simulink model "gm_PMLSM_FOC_FixedPoint_vnl"  (R2026b)
settings: Solver=FixedStepDiscrete  StopTime=0.0063  FixedStep=2e-08
undefined symbols (not defined in the file): FOC_Fixed_Config, Lookup, Ts_ACR
libraries: hdlmdlgenlib x38, simulink x16, mcbeeMathTransformLib x2
(part 1 of 6)
settings Model: Creator=lww  LastModifiedBy=lww
settings DataIOCC: ExternalInput=M3_HDL_Stimulus  LoadExternalInput=on
settings OptimizationCC: BlockReduction=off  ConditionallyExecuteInputs=off  DefaultParameterBehavior=Inlined
settings DebuggingCC: FixptConstOverflowMsg=error  InheritedTsInSrcMsg=none  IntegerOverflowMsg=error  IntegerSaturationMsg=error

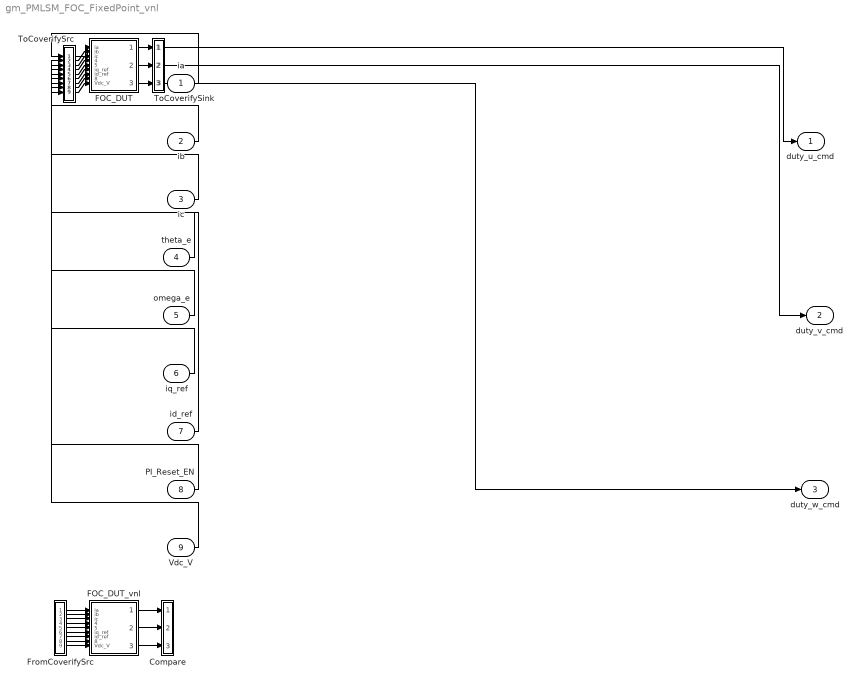
== system gm_PMLSM_FOC_FixedPoint_vnl ==
  ia : Inport  OutDataTypeStr=FOC_Fixed_Config.Types.Current  SampleTime=Ts_ACR  Interpolate=off
  ib : Inport  Port=2  OutDataTypeStr=FOC_Fixed_Config.Types.Current  SampleTime=Ts_ACR  Interpolate=off
  ic : Inport  Port=3  OutDataTypeStr=FOC_Fixed_Config.Types.Current  SampleTime=Ts_ACR  Interpolate=off
  theta_e : Inport  Port=4  OutDataTypeStr=FOC_Fixed_Config.Types.Angle  SampleTime=Ts_ACR  Interpolate=off
  omega_e : Inport  Port=5  OutDataTypeStr=FOC_Fixed_Config.Types.Omega  SampleTime=Ts_ACR  Interpolate=off
  iq_ref : Inport  Port=6  OutDataTypeStr=FOC_Fixed_Config.Types.Current  SampleTime=Ts_ACR  Interpolate=off
  id_ref : Inport  Port=7  OutDataTypeStr=FOC_Fixed_Config.Types.Current  SampleTime=Ts_ACR  Interpolate=off
  PI_Reset_EN : Inport  Port=8  OutDataTypeStr=boolean  SampleTime=Ts_ACR  Interpolate=off
  Vdc_V : Inport  Port=9  OutDataTypeStr=FOC_Fixed_Config.Types.Bus  SampleTime=Ts_ACR  Interpolate=off
  Compare : Subsystem
      mask Display: disp('')
  FOC_DUT : Subsystem
  FOC_DUT_vnl : Subsystem  TreatAsAtomicUnit=on
  FromCoverifySrc : Subsystem
      mask Display: disp('')
  ToCoverifySink : Subsystem
      mask Display: disp('')
  ToCoverifySrc : Subsystem
      mask Display: disp('')
  duty_u_cmd : Outport  OutDataTypeStr=FOC_Fixed_Config.Types.Duty
  duty_v_cmd : Outport  Port=2  OutDataTypeStr=FOC_Fixed_Config.Types.Duty
  duty_w_cmd : Outport  Port=3  OutDataTypeStr=FOC_Fixed_Config.Types.Duty
  wires:
  ToCoverifySrc/1(out1) -> FOC_DUT/1(ia)
  ToCoverifySrc/2(out2) -> FOC_DUT/2(ib)
  ToCoverifySrc/3(out3) -> FOC_DUT/3(ic)
  ToCoverifySrc/4(out4) -> FOC_DUT/4(theta_e)
  ToCoverifySrc/5(out5) -> FOC_DUT/5(omega_e)
  ToCoverifySrc/6(out6) -> FOC_DUT/6(iq_ref)
  ToCoverifySrc/7(out7) -> FOC_DUT/7(id_ref)
  ToCoverifySrc/8(out8) -> FOC_DUT/8(PI_Reset_EN)
  ToCoverifySrc/9(out9) -> FOC_DUT/9(Vdc_V)
  FOC_DUT/1(duty_u_cmd) -> ToCoverifySink/1(in1)
  FOC_DUT/2(duty_v_cmd) -> ToCoverifySink/2(in2)
  FOC_DUT/3(duty_w_cmd) -> ToCoverifySink/3(in3)
  ia/1 -> ToCoverifySrc/1(in1)
  ib/1 -> ToCoverifySrc/2(in2)
  ic/1 -> ToCoverifySrc/3(in3)
  theta_e/1 -> ToCoverifySrc/4(in4)
  omega_e/1 -> ToCoverifySrc/5(in5)
  iq_ref/1 -> ToCoverifySrc/6(in6)
  id_ref/1 -> ToCoverifySrc/7(in7)
  PI_Reset_EN/1 -> ToCoverifySrc/8(in8)
  Vdc_V/1 -> ToCoverifySrc/9(in9)
  ToCoverifySink/1(out1) -> duty_u_cmd/1
  ToCoverifySink/2(out2) -> duty_v_cmd/1
  ToCoverifySink/3(out3) -> duty_w_cmd/1
  FromCoverifySrc/1(out1) -> FOC_DUT_vnl/1(ia)
  FromCoverifySrc/2(out2) -> FOC_DUT_vnl/2(ib)
  FromCoverifySrc/3(out3) -> FOC_DUT_vnl/3(ic)
  FromCoverifySrc/4(out4) -> FOC_DUT_vnl/4(theta_e)
  FromCoverifySrc/5(out5) -> FOC_DUT_vnl/5(omega_e)
  FromCoverifySrc/6(out6) -> FOC_DUT_vnl/6(iq_ref)
  FromCoverifySrc/7(out7) -> FOC_DUT_vnl/7(id_ref)
  FromCoverifySrc/8(out8) -> FOC_DUT_vnl/8(PI_Reset_EN)
  FromCoverifySrc/9(out9) -> FOC_DUT_vnl/9(Vdc_V)
  FOC_DUT_vnl/1(duty_u_cmd) -> Compare/1(in1)
  FOC_DUT_vnl/2(duty_v_cmd) -> Compare/2(in2)
  FOC_DUT_vnl/3(duty_w_cmd) -> Compare/3(in3)

== system gm_PMLSM_FOC_FixedPoint_vnl/Compare ==
  in1 : Inport
  in2 : Inport  Port=2
  in3 : Inport  Port=3
  Assert_duty_u_cmd : Subsystem
  Assert_duty_v_cmd : Subsystem
  Assert_duty_w_cmd : Subsystem
  CleanupScopes : Subsystem
      settings: OpenFcn=|
      | blkName = gcb; %self block
      | idx = regexp(blkName, '/CleanupScopes$', 'once');
      | blkParent = blkName(1:idx-1);
      | blks=find_system(blkParent, 'LookUnderMasks', 'all','blocktype', 'Scope');
      | for itr = 1:length(blks)
      | 	 hScopeCfg = get_param(blks{itr},'ScopeConfiguration');
      | 	 hScopeCfg.Visible = ~ hScopeCfg.Visible;
      | end
      | drawnow;
      mask Display: fprintf(message('hdlcoder:cosim:vnl_dblclick').getString());
  Enable : Subsystem
      settings: OpenFcn=|
      | blkName = gcb;
      | idx = regexp(blkName, '/Enable$', 'once');
      | blkParent = blkName(1:idx-1);
      | blks=find_system(blkParent, 'LookUnderMasks', 'all','blocktype', 'Assertion');
      | e = get_param(blks{1}, 'Enabled');
      | if strcmp(e, 'on'), f= 'off';, else, f = 'on';, end
      | for ii=1:length(blks), set_param(blks{ii}, 'Enabled', f);, end
      | set_param(gcb, 'MaskDisplay',['fprintf(message(''hdlcoder:cosim:vnl_dblclick_assertions'',','''',upper(e),'''',').getString())']);
      mask Display: fprintf(message('hdlcoder:cosim:vnl_dblclick_assertions','OFF').getString());
  pathdelay1 : Delay  DelayLength=1
  pathdelay2 : Delay  DelayLength=1
  pathdelay3 : Delay  DelayLength=1
  wires:
  in1/1 -> pathdelay1/1
  pathdelay1/1 -> Assert_duty_u_cmd/1(cosim)
  [out1] -> Assert_duty_u_cmd/2(dut)
  in2/1 -> pathdelay2/1
  pathdelay2/1 -> Assert_duty_v_cmd/1(cosim)
  [out2] -> Assert_duty_v_cmd/2(dut)
  in3/1 -> pathdelay3/1
  pathdelay3/1 -> Assert_duty_w_cmd/1(cosim)
  [out3] -> Assert_duty_w_cmd/2(dut)

== system gm_PMLSM_FOC_FixedPoint_vnl/FOC_DUT ==
  ia : Inport  OutDataTypeStr=fixdt(1, 32, 24)  PortDimensions=1  SampleTime=0.0001
  ib : Inport  Port=2  OutDataTypeStr=fixdt(1, 32, 24)  PortDimensions=1  SampleTime=0.0001
  ic : Inport  Port=3  OutDataTypeStr=fixdt(1, 32, 24)  PortDimensions=1  SampleTime=0.0001
  theta_e : Inport  Port=4  OutDataTypeStr=fixdt(1, 40, 32)  PortDimensions=1  SampleTime=0.0001
  omega_e : Inport  Port=5  OutDataTypeStr=fixdt(1, 40, 24)  PortDimensions=1  SampleTime=0.0001
  iq_ref : Inport  Port=6  OutDataTypeStr=fixdt(1, 32, 24)  PortDimensions=1  SampleTime=0.0001
  id_ref : Inport  Port=7  OutDataTypeStr=fixdt(1, 32, 24)  PortDimensions=1  SampleTime=0.0001
  PI_Reset_EN : Inport  Port=8  OutDataTypeStr=boolean  PortDimensions=1  SampleTime=0.0001
  Vdc_V : Inport  Port=9  OutDataTypeStr=fixdt(0, 32, 24)  PortDimensions=1  SampleTime=0.0001
  FOC_DUT : Subsystem  TreatAsAtomicUnit=on
  t : RateTransition  OutPortSampleTimeOpt=Multiple of input port sample time  OutPortSampleTimeMultiple=5000
  t1 : RateTransition  OutPortSampleTimeOpt=Multiple of input port sample time  OutPortSampleTimeMultiple=5000
  t2 : RateTransition  OutPortSampleTimeOpt=Multiple of input port sample time  OutPortSampleTimeMultiple=5000
  duty_u_cmd : Outport  OutDataTypeStr=fixdt(0, 32, 30)  PortDimensions=1  SampleTime=0.0001
  duty_v_cmd : Outport  Port=2  OutDataTypeStr=fixdt(0, 32, 30)  PortDimensions=1  SampleTime=0.0001
  duty_w_cmd : Outport  Port=3  OutDataTypeStr=fixdt(0, 32, 30)  PortDimensions=1  SampleTime=0.0001
  wires:
  t2/1 -> duty_w_cmd/1
  t1/1 -> duty_v_cmd/1
  t/1 -> duty_u_cmd/1
  FOC_DUT/3(duty_w_cmd) -> t2/1
  FOC_DUT/1(duty_u_cmd) -> t/1
  Vdc_V/1 -> FOC_DUT/9(Vdc_V)
  FOC_DUT/2(duty_v_cmd) -> t1/1
  PI_Reset_EN/1 -> FOC_DUT/8(PI_Reset_EN)
  ib/1 -> FOC_DUT/2(ib)
  ia/1 -> FOC_DUT/1(ia)
  ic/1 -> FOC_DUT/3(ic)
  theta_e/1 -> FOC_DUT/4(theta_e)
  omega_e/1 -> FOC_DUT/5(omega_e)
  iq_ref/1 -> FOC_DUT/6(iq_ref)
  id_ref/1 -> FOC_DUT/7(id_ref)

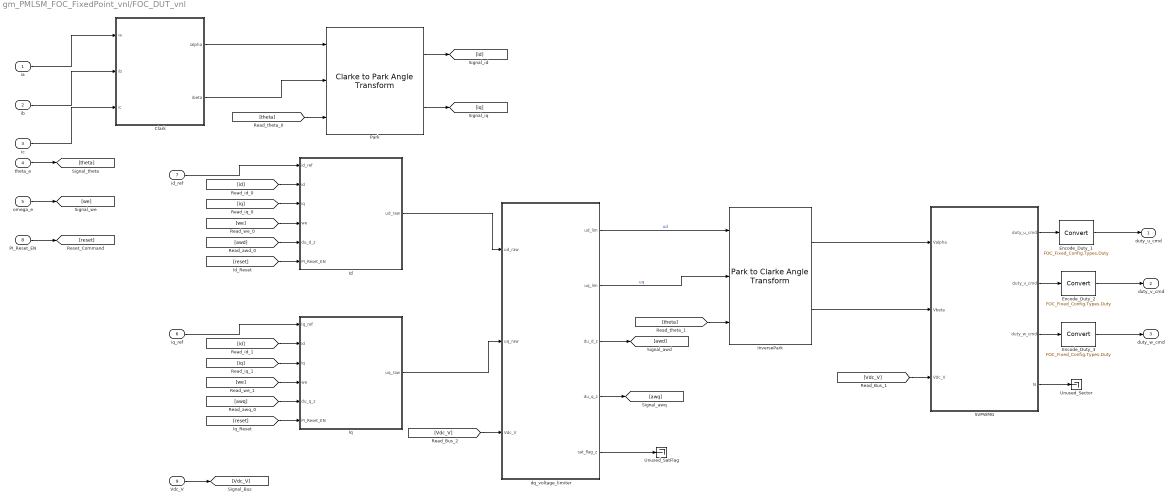
== system gm_PMLSM_FOC_FixedPoint_vnl/FOC_DUT_vnl ==
  ia : Inport
  ib : Inport  Port=2
  ic : Inport  Port=3
  theta_e : Inport  Port=4
  omega_e : Inport  Port=5
  iq_ref : Inport  Port=6
  id_ref : Inport  Port=7
  PI_Reset_EN : Inport  Port=8
  Vdc_V : Inport  Port=9
  Clark : Subsystem  TreatAsAtomicUnit=on  RTWFcnName=Clack_Fun
      settings: RTWFcnNameOpts=User specified
  Encode_Duty_1 : DataTypeConversion  OutDataTypeStr=FOC_Fixed_Config.Types.Duty  RndMeth=Convergent
  Encode_Duty_2 : DataTypeConversion  OutDataTypeStr=FOC_Fixed_Config.Types.Duty  RndMeth=Convergent
  Encode_Duty_3 : DataTypeConversion  OutDataTypeStr=FOC_Fixed_Config.Types.Duty  RndMeth=Convergent
  Id : Subsystem  TreatAsAtomicUnit=on  RTWFcnName=Id_Fun
      settings: RTWFcnNameOpts=User specified
  InversePark : mcbeeMathTransformLib/Park to Clarke Angle Transform  AxisAlignment=D-axis  UseWithEmbedded=on  PhaseInput=Two inputs  ThetaInput=Electrical position  AngleInput=Radians  N_points=1024
      settings: LibrarySourceBlock=mcbhdllib/Controls/Math Transforms/Inverse Park Transform
  Iq : Subsystem  TreatAsAtomicUnit=on  RTWFcnName=Iq_Fun
      settings: RTWFcnNameOpts=User specified
  Park : mcbeeMathTransformLib/Clarke to Park Angle Transform  AxisAlignment=D-axis  UseWithEmbedded=on  PhaseInput=Two inputs  ThetaInput=Electrical position  AngleInput=Radians  N_points=1024
      settings: LibrarySourceBlock=mcblib/Controls/Math Transforms/Park Transform
  SVPWMG : Subsystem  TreatAsAtomicUnit=on  RTWFcnName=SVPWM_Gen_Fun
      settings: RTWFcnNameOpts=User specified
  Unused_SatFlag : Terminator
  Unused_Sector : Terminator
  dq_voltage_limiter : Subsystem
  duty_u_cmd : Outport
  duty_v_cmd : Outport  Port=2
  duty_w_cmd : Outport  Port=3
  wires:
  dq_voltage_limiter/3(du_d_z) -> [awd]
  dq_voltage_limiter/5(sat_flag_z) -> Unused_SatFlag/1
  dq_voltage_limiter/4(du_q_z) -> [awq]
  dq_voltage_limiter/2(uq_lim) -> InversePark/2  "uq"
  dq_voltage_limiter/1(ud_lim) -> InversePark/1  "ud"
  SVPWMG/4("N ") -> Unused_Sector/1
  SVPWMG/3(duty_w_cmd) -> Encode_Duty_3/1
  SVPWMG/2(duty_v_cmd) -> Encode_Duty_2/1
  SVPWMG/1(duty_u_cmd) -> Encode_Duty_1/1
  [we] -> Iq/4(we)
  [we] -> Id/4(we)
  [theta] -> InversePark/3
  [theta] -> Park/3
  [iq] -> Iq/3(iq)
  [iq] -> Id/3(iq)
  [id] -> Iq/2(id)
  [id] -> Id/2(id)
  [awq] -> Iq/5(du_q_z)
  [awd] -> Id/5(du_d_z)
  [Vdc_V] -> dq_voltage_limiter/3(Vdc_V)
  [Vdc_V] -> SVPWMG/3(Vdc_V)
  Park/2 -> [iq]
  Park/1 -> [id]
  [reset] -> Iq/6(PI_Reset_EN)
  Iq/1(uq_raw) -> dq_voltage_limiter/2(uq_raw)
  InversePark/2 -> SVPWMG/2(Vbeta)
  InversePark/1 -> SVPWMG/1(Valpha)
  [reset] -> Id/6(PI_Reset_EN)
  Id/1(ud_raw) -> dq_voltage_limiter/1(ud_raw)
  Encode_Duty_3/1 -> duty_w_cmd/1
  Encode_Duty_2/1 -> duty_v_cmd/1
  Encode_Duty_1/1 -> duty_u_cmd/1
  Clark/2(ibeta) -> Park/2
  Clark/1(ialpha) -> Park/1
  Vdc_V/1 -> [Vdc_V]
  PI_Reset_EN/1 -> [reset]
  id_ref/1 -> Id/1(id_ref)
  iq_ref/1 -> Iq/1(Iq_ref)
  omega_e/1 -> [we]
  theta_e/1 -> [theta]
  ic/1 -> Clark/3(ic)
  ib/1 -> Clark/2(ib)
  ia/1 -> Clark/1(ia)

== system gm_PMLSM_FOC_FixedPoint_vnl/FromCoverifySrc ==
  out1 : Outport
  out2 : Outport  Port=2
  out3 : Outport  Port=3
  out4 : Outport  Port=4
  out5 : Outport  Port=5
  out6 : Outport  Port=6
  out7 : Outport  Port=7
  out8 : Outport  Port=8
  out9 : Outport  Port=9
  wires:
  [in1] -> out1/1
  [in2] -> out2/1
  [in3] -> out3/1
  [in4] -> out4/1
  [in5] -> out5/1
  [in6] -> out6/1
  [in7] -> out7/1
  [in8] -> out8/1
  [in9] -> out9/1

== system gm_PMLSM_FOC_FixedPoint_vnl/ToCoverifySink ==
  in1 : Inport
  in2 : Inport  Port=2
  in3 : Inport  Port=3
  out1 : Outport
  out2 : Outport  Port=2
  out3 : Outport  Port=3
  tag scope: out1=global, out2=global, out3=global
  wires:
  in1/1 -> out1/1, [out1]
  in2/1 -> out2/1, [out2]
  in3/1 -> out3/1, [out3]

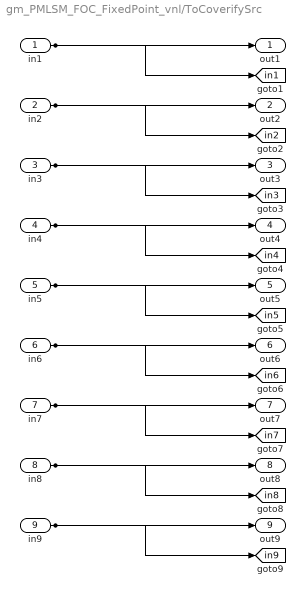
== system gm_PMLSM_FOC_FixedPoint_vnl/ToCoverifySrc ==
  in1 : Inport
  in2 : Inport  Port=2
  in3 : Inport  Port=3
  in4 : Inport  Port=4
  in5 : Inport  Port=5
  in6 : Inport  Port=6
  in7 : Inport  Port=7
  in8 : Inport  Port=8
  in9 : Inport  Port=9
  out1 : Outport
  out2 : Outport  Port=2
  out3 : Outport  Port=3
  out4 : Outport  Port=4
  out5 : Outport  Port=5
  out6 : Outport  Port=6
  out7 : Outport  Port=7
  out8 : Outport  Port=8
  out9 : Outport  Port=9
  tag scope: in1=global, in2=global, in3=global, in4=global, in5=global, in6=global, in7=global, in8=global, in9=global
  wires:
  in1/1 -> out1/1, [in1]
  in2/1 -> out2/1, [in2]
  in3/1 -> out3/1, [in3]
  in4/1 -> out4/1, [in4]
  in5/1 -> out5/1, [in5]
  in6/1 -> out6/1, [in6]
  in7/1 -> out7/1, [in7]
  in8/1 -> out8/1, [in8]
  in9/1 -> out9/1, [in9]

== system gm_PMLSM_FOC_FixedPoint_vnl/Compare/Assert_duty_u_cmd ==
  cosim : Inport
  dut : Inport  Port=2
  AssertEq : Assertion  StopWhenAssertionFail=off
  Compare To Zero : simulink/Logic and Bit Operations/Compare To Zero  relop===  OutDataTypeStr=boolean
  Constant1 : Constant  Value=0  OutDataTypeStr=fixdt(0, 32, 30)  SampleTime=-1
  Counter : simulink/Sources/Counter Free-Running  NumBits=32  tsamp=-1
  IgnoreCycles : Constant  Value=2  SampleTime=-1
  Relational Operator : RelationalOperator  Operator=<  OutDataTypeStr=boolean  InputSameDT=off
  Relational Operator1 : RelationalOperator  Operator===  OutDataTypeStr=boolean  InputSameDT=off
  Switch : Switch  Criteria=u2 ~= 0  SaturateOnIntegerOverflow=off  InputSameDT=off
  Switch1 : Switch  Criteria=u2 ~= 0  SaturateOnIntegerOverflow=off  InputSameDT=off
  compare: duty_u_cmd : Scope  NumInputPorts=3
      settings: ActiveDisplayYMinimum=-5  ActiveDisplayYMaximum=5  DataLoggingVariableName=ScopeData3
  wires:
  Compare To Zero/1 -> compare: duty_u_cmd/3  "err"
  Relational Operator1/1 -> Compare To Zero/1, AssertEq/1
  Switch1/1 -> compare: duty_u_cmd/1, Relational Operator1/1
  Switch/1 -> compare: duty_u_cmd/2, Relational Operator1/2
  Constant1/1 -> Switch/1, Switch1/1
  Relational Operator/1 -> Switch/2, Switch1/2
  cosim/1 -> Switch1/3  "cosim"
  dut/1 -> Switch/3  "dut ref"
  Counter/1 -> Relational Operator/1
  IgnoreCycles/1 -> Relational Operator/2

== system gm_PMLSM_FOC_FixedPoint_vnl/Compare/Assert_duty_v_cmd ==
  cosim : Inport
  dut : Inport  Port=2
  AssertEq : Assertion  StopWhenAssertionFail=off
  Compare To Zero : simulink/Logic and Bit Operations/Compare To Zero  relop===  OutDataTypeStr=boolean
  Constant1 : Constant  Value=0  OutDataTypeStr=fixdt(0, 32, 30)  SampleTime=-1
  Counter : simulink/Sources/Counter Free-Running  NumBits=32  tsamp=-1
  IgnoreCycles : Constant  Value=2  SampleTime=-1
  Relational Operator : RelationalOperator  Operator=<  OutDataTypeStr=boolean  InputSameDT=off
  Relational Operator1 : RelationalOperator  Operator===  OutDataTypeStr=boolean  InputSameDT=off
  Switch : Switch  Criteria=u2 ~= 0  SaturateOnIntegerOverflow=off  InputSameDT=off
  Switch1 : Switch  Criteria=u2 ~= 0  SaturateOnIntegerOverflow=off  InputSameDT=off
  compare: duty_v_cmd : Scope  NumInputPorts=3
      settings: ActiveDisplayYMinimum=-5  ActiveDisplayYMaximum=5  DataLoggingVariableName=ScopeData3
  wires:
  Compare To Zero/1 -> compare: duty_v_cmd/3  "err"
  Relational Operator1/1 -> Compare To Zero/1, AssertEq/1
  Switch1/1 -> compare: duty_v_cmd/1, Relational Operator1/1
  Switch/1 -> compare: duty_v_cmd/2, Relational Operator1/2
  Constant1/1 -> Switch/1, Switch1/1
  Relational Operator/1 -> Switch/2, Switch1/2
  cosim/1 -> Switch1/3  "cosim"
  dut/1 -> Switch/3  "dut ref"
  Counter/1 -> Relational Operator/1
  IgnoreCycles/1 -> Relational Operator/2

== system gm_PMLSM_FOC_FixedPoint_vnl/Compare/Assert_duty_w_cmd ==
  cosim : Inport
  dut : Inport  Port=2
  AssertEq : Assertion  StopWhenAssertionFail=off
  Compare To Zero : simulink/Logic and Bit Operations/Compare To Zero  relop===  OutDataTypeStr=boolean
  Constant1 : Constant  Value=0  OutDataTypeStr=fixdt(0, 32, 30)  SampleTime=-1
  Counter : simulink/Sources/Counter Free-Running  NumBits=32  tsamp=-1
  IgnoreCycles : Constant  Value=2  SampleTime=-1
  Relational Operator : RelationalOperator  Operator=<  OutDataTypeStr=boolean  InputSameDT=off
  Relational Operator1 : RelationalOperator  Operator===  OutDataTypeStr=boolean  InputSameDT=off
  Switch : Switch  Criteria=u2 ~= 0  SaturateOnIntegerOverflow=off  InputSameDT=off
  Switch1 : Switch  Criteria=u2 ~= 0  SaturateOnIntegerOverflow=off  InputSameDT=off
  compare: duty_w_cmd : Scope  NumInputPorts=3
      settings: ActiveDisplayYMinimum=-5  ActiveDisplayYMaximum=5  DataLoggingVariableName=ScopeData3
  wires:
  Compare To Zero/1 -> compare: duty_w_cmd/3  "err"
  Relational Operator1/1 -> Compare To Zero/1, AssertEq/1
  Switch1/1 -> compare: duty_w_cmd/1, Relational Operator1/1
  Switch/1 -> compare: duty_w_cmd/2, Relational Operator1/2
  Constant1/1 -> Switch/1, Switch1/1
  Relational Operator/1 -> Switch/2, Switch1/2
  cosim/1 -> Switch1/3  "cosim"
  dut/1 -> Switch/3  "dut ref"
  Counter/1 -> Relational Operator/1
  IgnoreCycles/1 -> Relational Operator/2

== system gm_PMLSM_FOC_FixedPoint_vnl/Compare/CleanupScopes ==

== system gm_PMLSM_FOC_FixedPoint_vnl/Compare/Enable ==

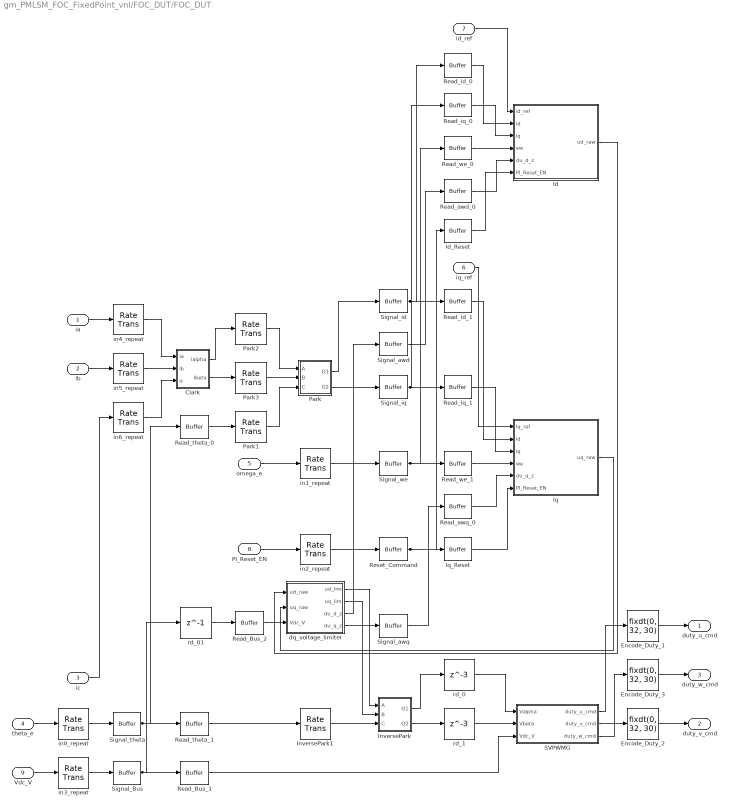
== system gm_PMLSM_FOC_FixedPoint_vnl/FOC_DUT/FOC_DUT ==
  ia : Inport  OutDataTypeStr=fixdt(1,32,24,'DataTypeOverride', 'Off')  PortDimensions=1  SampleTime=0.0001
  ib : Inport  Port=2  OutDataTypeStr=fixdt(1,32,24,'DataTypeOverride', 'Off')  PortDimensions=1  SampleTime=0.0001
  ic : Inport  Port=3  OutDataTypeStr=fixdt(1,32,24,'DataTypeOverride', 'Off')  PortDimensions=1  SampleTime=0.0001
  theta_e : Inport  Port=4  OutDataTypeStr=fixdt(1,40,32,'DataTypeOverride', 'Off')  PortDimensions=1  SampleTime=0.0001
  omega_e : Inport  Port=5  OutDataTypeStr=fixdt(1,40,24,'DataTypeOverride', 'Off')  PortDimensions=1  SampleTime=0.0001
  iq_ref : Inport  Port=6  OutDataTypeStr=fixdt(1,32,24,'DataTypeOverride', 'Off')  PortDimensions=1  SampleTime=0.0001
  id_ref : Inport  Port=7  OutDataTypeStr=fixdt(1,32,24,'DataTypeOverride', 'Off')  PortDimensions=1  SampleTime=0.0001
  PI_Reset_EN : Inport  Port=8  OutDataTypeStr=boolean  PortDimensions=1  SampleTime=0.0001
  Vdc_V : Inport  Port=9  OutDataTypeStr=fixdt(0,32,24,'DataTypeOverride', 'Off')  PortDimensions=1  SampleTime=0.0001
  Clark : Subsystem
  Encode_Duty_1 : DataTypeConversion  OutDataTypeStr=fixdt(0, 32, 30)  RndMeth=Convergent  SampleTime=2e-08
  Encode_Duty_2 : DataTypeConversion  OutDataTypeStr=fixdt(0, 32, 30)  RndMeth=Convergent  SampleTime=2e-08
  Encode_Duty_3 : DataTypeConversion  OutDataTypeStr=fixdt(0, 32, 30)  RndMeth=Convergent  SampleTime=2e-08
  Id : Subsystem
  Id_Reset : hdlmdlgenlib/Buffer
  InversePark : Subsystem  mask(Park to Clarke Angle Transform){AxisAlignment=D-axis, UseWithEmbedded=on, PhaseInput='Two inputs', ThetaInput=Electrical position, AngleInput=Radians, N_points=1024}
      mask prompts: AxisAlignment "shared_mcbeeblks:mcbeeblks:InvPBlkPrmAlign"; UseWithEmbedded "shared_mcbeeblks:mcbeeblks:BlkEmbeddedUse"; PhaseInput "shared_mcbeeblks:mcbeeblks:InvPPrmInp"; ThetaInput "shared_mcbeeblks:mcbeeblks:InvPPrmTheta"; AngleInput "shared_mcbeeblks:mcbeeblks:InvPThetaUnits"; N_points "shared_mcbeeblks:mcbeeblks:InvPPrmLUTSize"
      mask help: shared_mcbeeblks:mcbeeblks:InvPBlkDlgDes
      mask init:
      | AngleInput = 2;
      | AxisAlignment = 1;
      | N_points = 1024;
      | PhaseInput = 1;
      | ThetaInput = 1;
      | UseWithEmbedded = 1;
      mask Help: eval('mcbeeutil.mcbeesharedhelp(''inverseparktransform'')')
      mask TypeOptions AxisAlignment: shared_mcbeeblks:mcbeeblks:InvPpopDaxis | shared_mcbeeblks:mcbeeblks:InvPpopQaxis
      mask Callback UseWithEmbedded: mcbeeutil.mcbeeParkToClarkeCb('embeddeduse',gcbh);
      mask TypeOptions ThetaInput: shared_mcbeeblks:mcbeeblks:InvPPopElec | shared_mcbeeblks:mcbeeblks:InvPPopSinCos
      mask Callback ThetaInput: mcbeeutil.mcbeeParkToClarkeCb('ThetaInputCb',gcbh);
      mask TypeOptions AngleInput: shared_mcbeeblks:mcbeeblks:InvPPopPUUnit | shared_mcbeeblks:mcbeeblks:InvPPopRadUnit | shared_mcbeeblks:mcbeeblks:InvPPopDegUnit
      mask Display:
      | fprintf('Park to\nClarke')
      | port_label('input',1, 'd','interpreter', 'tex');
      | port_label('input',2, 'q','interpreter', 'tex');
      | port_label('input',3, '\theta_e','interpreter', 'tex');
      | port_label('output',1, '\alpha','interpreter', 'tex');
      | port_label('output',2, '\beta','interpreter', 'tex');
  InversePark1 : RateTransition  OutPortSampleTimeOpt=Multiple of input port sample time  OutPortSampleTimeMultiple=5000
  Iq : Subsystem
  Iq_Reset : hdlmdlgenlib/Buffer
  Park : Subsystem  mask(Clarke to Park Angle Transform){AxisAlignment=D-axis, UseWithEmbedded=on, PhaseInput='Two inputs', ThetaInput=Electrical position, AngleInput=Radians, N_points=1024}
      mask prompts: AxisAlignment "shared_mcbeeblks:mcbeeblks:ParkBlkPrmAlign"; UseWithEmbedded "shared_mcbeeblks:mcbeeblks:BlkEmbeddedUse"; PhaseInput "shared_mcbeeblks:mcbeeblks:ParkPrmInp"; ThetaInput "shared_mcbeeblks:mcbeeblks:ParkPrmTheta"; AngleInput "shared_mcbeeblks:mcbeeblks:ParkPrmThetaUnits"; N_points "shared_mcbeeblks:mcbeeblks:ParkPrmLUTSize"
      mask help: shared_mcbeeblks:mcbeeblks:ParkBlkDlgDes
      mask init:
      | AngleInput = 2;
      | AxisAlignment = 1;
      | N_points = 1024;
      | PhaseInput = 1;
      | ThetaInput = 1;
      | UseWithEmbedded = 1;
      mask Help: eval('mcbeeutil.mcbeesharedhelp(''parktransform'')')
      mask TypeOptions AxisAlignment: shared_mcbeeblks:mcbeeblks:ParkpopDaxis | shared_mcbeeblks:mcbeeblks:ParkpopQaxis
      mask Callback UseWithEmbedded: mcbeeutil.mcbeeClarkeToParkCb('embeddeduse',gcbh);
      mask TypeOptions ThetaInput: shared_mcbeeblks:mcbeeblks:ParkPopElec | shared_mcbeeblks:mcbeeblks:ParkPopSinCos
      mask Callback ThetaInput: mcbeeutil.mcbeeClarkeToParkCb('ThetaInputCb',gcbh)
      mask TypeOptions AngleInput: shared_mcbeeblks:mcbeeblks:ParkPopPUUnit | shared_mcbeeblks:mcbeeblks:ParkPopRadUnit | shared_mcbeeblks:mcbeeblks:ParkPopDegUnit
      mask Display:
      | fprintf('Clarke to\nPark')
      | port_label('input',1, '\alpha','interpreter', 'tex');
      | port_label('input',2, '\beta','interpreter', 'tex');
      | port_label('input',3, '\theta_e','interpreter', 'tex');
      | port_label('output',1, 'd','interpreter', 'tex');
      | port_label('output',2, 'q','interpreter', 'tex');
  Park1 : RateTransition  OutPortSampleTimeOpt=Multiple of input port sample time  OutPortSampleTimeMultiple=5000
  Park2 : RateTransition  OutPortSampleTimeOpt=Multiple of input port sample time  OutPortSampleTimeMultiple=5000
  Park3 : RateTransition  OutPortSampleTimeOpt=Multiple of input port sample time  OutPortSampleTimeMultiple=5000
  Read_Bus_1 : hdlmdlgenlib/Buffer
  Read_Bus_2 : hdlmdlgenlib/Buffer
  Read_awd_0 : hdlmdlgenlib/Buffer
  Read_awq_0 : hdlmdlgenlib/Buffer
  Read_id_0 : hdlmdlgenlib/Buffer
  Read_id_1 : hdlmdlgenlib/Buffer
  Read_iq_0 : hdlmdlgenlib/Buffer
  Read_iq_1 : hdlmdlgenlib/Buffer
  Read_theta_0 : hdlmdlgenlib/Buffer
  Read_theta_1 : hdlmdlgenlib/Buffer
  Read_we_0 : hdlmdlgenlib/Buffer
  Read_we_1 : hdlmdlgenlib/Buffer
  Reset_Command : hdlmdlgenlib/Buffer
  SVPWMG : Subsystem
  Signal_Bus : hdlmdlgenlib/Buffer
  Signal_awd : hdlmdlgenlib/Buffer
  Signal_awq : hdlmdlgenlib/Buffer
  Signal_id : hdlmdlgenlib/Buffer
  Signal_iq : hdlmdlgenlib/Buffer
  Signal_theta : hdlmdlgenlib/Buffer
  Signal_we : hdlmdlgenlib/Buffer
  dq_voltage_limiter : Subsystem
  in0_repeat : RateTransition  Integrity=off  Deterministic=off  OutPortSampleTimeOpt=Multiple of input port sample time  OutPortSampleTimeMultiple=1/5000
  in1_repeat : RateTransition  Integrity=off  Deterministic=off  OutPortSampleTimeOpt=Multiple of input port sample time  OutPortSampleTimeMultiple=1/5000
  in2_repeat : RateTransition  Integrity=off  Deterministic=off  OutPortSampleTimeOpt=Multiple of input port sample time  OutPortSampleTimeMultiple=1/5000
  in3_repeat : RateTransition  Integrity=off  Deterministic=off  OutPortSampleTimeOpt=Multiple of input port sample time  OutPortSampleTimeMultiple=1/5000
  in4_repeat : RateTransition  Integrity=off  Deterministic=off  OutPortSampleTimeOpt=Multiple of input port sample time  OutPortSampleTimeMultiple=1/5000
  in5_repeat : RateTransition  Integrity=off  Deterministic=off  OutPortSampleTimeOpt=Multiple of input port sample time  OutPortSampleTimeMultiple=1/5000
  in6_repeat : RateTransition  Integrity=off  Deterministic=off  OutPortSampleTimeOpt=Multiple of input port sample time  OutPortSampleTimeMultiple=1/5000
  rd_0 : Delay  DelayLength=3  InitialCondition=0  SampleTime=2e-08
  rd_01 : Delay  DelayLength=1  InitialCondition=0  SampleTime=2e-08
  rd_1 : Delay  DelayLength=3  InitialCondition=0  SampleTime=2e-08
  duty_u_cmd : Outport  OutDataTypeStr=fixdt(0,32,30,'DataTypeOverride', 'Off')  PortDimensions=1  SampleTime=2e-08
  duty_v_cmd : Outport  Port=2  OutDataTypeStr=fixdt(0,32,30,'DataTypeOverride', 'Off')  PortDimensions=1  SampleTime=2e-08
  duty_w_cmd : Outport  Port=3  OutDataTypeStr=fixdt(0,32,30,'DataTypeOverride', 'Off')  PortDimensions=1  SampleTime=2e-08
  wires:
  Encode_Duty_3/1 -> duty_w_cmd/1
  Iq/1(uq_raw) -> dq_voltage_limiter/2(uq_raw)
  Read_awq_0/1 -> Iq/5(du_q_z)
  Read_iq_1/1 -> Iq/3(iq)
  Read_id_1/1 -> Iq/2(id)
  rd_0/1 -> SVPWMG/1(Valpha)
  iq_ref/1 -> Iq/1(Iq_ref)
  Read_we_0/1 -> Id/4(we)
  Read_iq_0/1 -> Id/3(iq)
  InversePark/1(O1) -> rd_0/1
  Signal_we/1 -> Read_we_0/1, Read_we_1/1
  Signal_iq/1 -> Read_iq_0/1, Read_iq_1/1
  Signal_awd/1 -> Read_awd_0/1
  InversePark1/1 -> InversePark/3(C)
  dq_voltage_limiter/4(du_q_z) -> Signal_awq/1
  SVPWMG/1(duty_u_cmd) -> Encode_Duty_1/1
  dq_voltage_limiter/3(du_d_z) -> Signal_awd/1
  Read_we_1/1 -> Iq/4(we)
  dq_voltage_limiter/1(ud_lim) -> InversePark/1(A)
  Encode_Duty_1/1 -> duty_u_cmd/1
  in2_repeat/1 -> Reset_Command/1
  in1_repeat/1 -> Signal_we/1
  Id_Reset/1 -> Id/6(PI_Reset_EN)
  Park/2(O2) -> Signal_iq/1
  SVPWMG/2(duty_v_cmd) -> Encode_Duty_2/1
  Park/1(O1) -> Signal_id/1
  Read_Bus_2/1 -> dq_voltage_limiter/3(Vdc_V)
  id_ref/1 -> Id/1(id_ref)
  PI_Reset_EN/1 -> in2_repeat/1
  omega_e/1 -> in1_repeat/1
  Park1/1 -> Park/3(C)
  Park3/1 -> Park/2(B)
  Park2/1 -> Park/1(A)
  Iq_Reset/1 -> Iq/6(PI_Reset_EN)
  Id/1(ud_raw) -> dq_voltage_limiter/1(ud_raw)
  Read_Bus_1/1 -> SVPWMG/3(Vdc_V)
  Read_theta_1/1 -> InversePark1/1
  rd_01/1 -> Read_Bus_2/1
  Signal_awq/1 -> Read_awq_0/1
  Encode_Duty_2/1 -> duty_v_cmd/1
  Read_theta_0/1 -> Park1/1
  InversePark/2(O2) -> rd_1/1
  Clark/2(ibeta) -> Park3/1
  Read_id_0/1 -> Id/2(id)
  Clark/1(ialpha) -> Park2/1
  Signal_theta/1 -> Read_theta_1/1, Read_theta_0/1
  in6_repeat/1 -> Clark/3(ic)
  Reset_Command/1 -> Id_Reset/1, Iq_Reset/1
  rd_1/1 -> SVPWMG/2(Vbeta)
  in5_repeat/1 -> Clark/2(ib)
  in4_repeat/1 -> Clark/1(ia)
  dq_voltage_limiter/2(uq_lim) -> InversePark/2(B)
  in0_repeat/1 -> Signal_theta/1
  Read_awd_0/1 -> Id/5(du_d_z)
  ic/1 -> in6_repeat/1
  Signal_Bus/1 -> rd_01/1, Read_Bus_1/1
  SVPWMG/3(duty_w_cmd) -> Encode_Duty_3/1
  ib/1 -> in5_repeat/1
  in3_repeat/1 -> Signal_Bus/1
  Vdc_V/1 -> in3_repeat/1
  ia/1 -> in4_repeat/1
  theta_e/1 -> in0_repeat/1
  Signal_id/1 -> Read_id_0/1, Read_id_1/1

== system gm_PMLSM_FOC_FixedPoint_vnl/FOC_DUT_vnl/Clark ==
  note: alpha=(A-0.5*(B+C))*2/3
      | Beta=sqrt(3)/2*(B-C)*2/3
  ia : Inport
  ib : Inport  Port=2
  ic : Inport  Port=3
  Add : Sum  Inputs=+--  OutDataTypeStr=FOC_Fixed_Config.Types.Work  AccumDataTypeStr=FOC_Fixed_Config.Types.Work  RndMeth=Convergent  SaturateOnIntegerOverflow=on
  Add1 : Sum  Inputs=+-  OutDataTypeStr=FOC_Fixed_Config.Types.Work  AccumDataTypeStr=FOC_Fixed_Config.Types.Work  RndMeth=Convergent  SaturateOnIntegerOverflow=on
  Gain : Gain  Gain=0.5  ParamDataTypeStr=FOC_Fixed_Config.Types.Coefficient  OutDataTypeStr=FOC_Fixed_Config.Types.Work  RndMeth=Convergent  SaturateOnIntegerOverflow=on
  Gain1 : Gain  Gain=0.5  ParamDataTypeStr=FOC_Fixed_Config.Types.Coefficient  OutDataTypeStr=FOC_Fixed_Config.Types.Work  RndMeth=Convergent  SaturateOnIntegerOverflow=on
  Gain2 : Gain  Gain=FOC_Fixed_Config.Coefficients.TwoThird.quantized  ParamDataTypeStr=FOC_Fixed_Config.Types.Coefficient  OutDataTypeStr=FOC_Fixed_Config.Types.Work  RndMeth=Convergent  SaturateOnIntegerOverflow=on
  Gain3 : Gain  Gain=FOC_Fixed_Config.Coefficients.InvSqrt3.quantized  ParamDataTypeStr=FOC_Fixed_Config.Types.Coefficient  OutDataTypeStr=FOC_Fixed_Config.Types.Work  RndMeth=Convergent  SaturateOnIntegerOverflow=on
  ialpha : Outport
  ibeta : Outport  Port=2
  wires:
  Gain/1 -> Add/2
  Gain2/1 -> ialpha/1  "ialf"
  Add/1 -> Gain2/1
  Gain3/1 -> ibeta/1  "ibeta"
  ic/1 -> Gain1/1, Add1/2
  Add1/1 -> Gain3/1
  ib/1 -> Gain/1, Add1/1
  ia/1 -> Add/1
  Gain1/1 -> Add/3

== system gm_PMLSM_FOC_FixedPoint_vnl/FOC_DUT_vnl/Id ==
  note: 起到使能时初始化一下的作用
  id_ref : Inport
  id : Inport  Port=2
  iq : Inport  Port=3
  we : Inport  Port=4
  du_d_z : Inport  Port=5
  PI_Reset_EN : Inport  Port=6
  " " : Gain  Gain=FOC_Fixed_Config.Coefficients.KiTs.quantized  ParamDataTypeStr=FOC_Fixed_Config.Types.Coefficient  OutDataTypeStr=FOC_Fixed_Config.Types.Work  RndMeth=Convergent  SaturateOnIntegerOverflow=on
  "  " : Gain  Gain=FOC_Fixed_Config.Coefficients.Kp.quantized  ParamDataTypeStr=FOC_Fixed_Config.Types.Coefficient  OutDataTypeStr=FOC_Fixed_Config.Types.Work  RndMeth=Convergent  SaturateOnIntegerOverflow=on
  Add1 : Sum  OutDataTypeStr=FOC_Fixed_Config.Types.Work  AccumDataTypeStr=FOC_Fixed_Config.Types.Work  RndMeth=Convergent  SaturateOnIntegerOverflow=on
  Add2 : Sum  Inputs=++-  OutDataTypeStr=FOC_Fixed_Config.Types.Work  AccumDataTypeStr=FOC_Fixed_Config.Types.Work  RndMeth=Convergent  SaturateOnIntegerOverflow=on
  Constant1 : Constant  Value=FOC_Fixed_Config.Coefficients.Lq.quantized  OutDataTypeStr=FOC_Fixed_Config.Types.Work
  Gain : Gain  Gain=FOC_Fixed_Config.Coefficients.Kaw_d.quantized  ParamDataTypeStr=FOC_Fixed_Config.Types.Coefficient  OutDataTypeStr=FOC_Fixed_Config.Types.Work  RndMeth=Convergent  SaturateOnIntegerOverflow=on
  Product : Product  OutDataTypeStr=FOC_Fixed_Config.Types.Work  RndMeth=Convergent  SaturateOnIntegerOverflow=on
  Product1 : Product  OutDataTypeStr=FOC_Fixed_Config.Types.Work  RndMeth=Convergent  SaturateOnIntegerOverflow=on
  Reset_Integral : Switch  Criteria=u2 > Threshold  Threshold=0.5  OutDataTypeStr=FOC_Fixed_Config.Types.Work  RndMeth=Convergent  InputSameDT=off
  Reset_Output : Switch  Criteria=u2 > Threshold  Threshold=0.5  OutDataTypeStr=FOC_Fixed_Config.Types.Work  RndMeth=Convergent  InputSameDT=off
  Reset_Zero : Constant  Value=0  OutDataTypeStr=FOC_Fixed_Config.Types.Work
  Sum : Sum  Inputs=|+-  OutDataTypeStr=FOC_Fixed_Config.Types.Work  AccumDataTypeStr=FOC_Fixed_Config.Types.Work  RndMeth=Convergent  SaturateOnIntegerOverflow=on
  Sum1 : Sum  Inputs=|+-  OutDataTypeStr=FOC_Fixed_Config.Types.Work  AccumDataTypeStr=FOC_Fixed_Config.Types.Work  RndMeth=Convergent  SaturateOnIntegerOverflow=on
  x_d_z : UnitDelay  SampleTime=-1
  ud_raw : Outport
  wires:
  [du_d_z] -> Gain/1
  [x_d_next] -> x_d_z/1
  du_d_z/1 -> [du_d_z]
  "  "/1 -> Add1/1
  Constant1/1 -> Product/2
  Product/1 -> Product1/1
  we/1 -> Product1/2
  Sum/1 -> "  "/1, " "/1
  id/1 -> Sum/2
  id_ref/1 -> Sum/1
  iq/1 -> Product/1
  Reset_Output/1 -> ud_raw/1
  Reset_Integral/1 -> [x_d_next]
  PI_Reset_EN/1 -> Reset_Output/2, Reset_Integral/2
  Reset_Zero/1 -> Reset_Output/1, Reset_Integral/1
  Add2/1 -> Reset_Integral/3  "x_d_next"
  Sum1/1 -> Reset_Output/3
  " "/1 -> Add2/2  "KiTs_q * e_d"
  Gain/1 -> Add2/3  "u_d,aw"
  x_d_z/1 -> Add2/1, Add1/2
  Add1/1 -> Sum1/1
  Product1/1 -> Sum1/2  "解耦项"

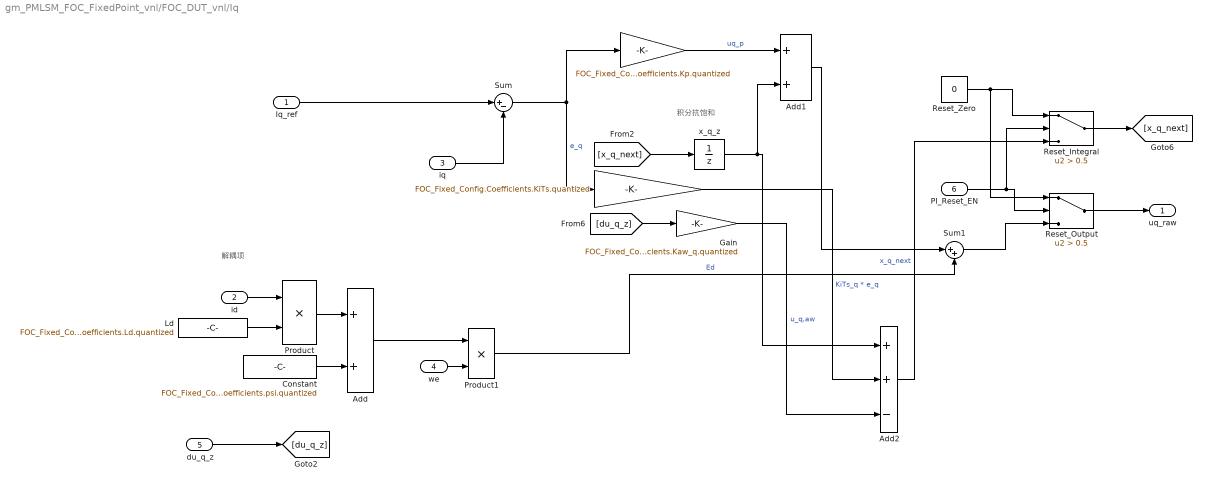
== system gm_PMLSM_FOC_FixedPoint_vnl/FOC_DUT_vnl/Iq ==
  note: 积分抗饱和
  note: 解耦项
  Iq_ref : Inport
  id : Inport  Port=2
  iq : Inport  Port=3
  we : Inport  Port=4
  du_q_z : Inport  Port=5
  PI_Reset_EN : Inport  Port=6
  " " : Gain  Gain=FOC_Fixed_Config.Coefficients.KiTs.quantized  ParamDataTypeStr=FOC_Fixed_Config.Types.Coefficient  OutDataTypeStr=FOC_Fixed_Config.Types.Work  RndMeth=Convergent  SaturateOnIntegerOverflow=on
  "  " : Gain  Gain=FOC_Fixed_Config.Coefficients.Kp.quantized  ParamDataTypeStr=FOC_Fixed_Config.Types.Coefficient  OutDataTypeStr=FOC_Fixed_Config.Types.Work  RndMeth=Convergent  SaturateOnIntegerOverflow=on
  Add : Sum  OutDataTypeStr=FOC_Fixed_Config.Types.Work  AccumDataTypeStr=FOC_Fixed_Config.Types.Work  RndMeth=Convergent  SaturateOnIntegerOverflow=on
  Add1 : Sum  OutDataTypeStr=FOC_Fixed_Config.Types.Work  AccumDataTypeStr=FOC_Fixed_Config.Types.Work  RndMeth=Convergent  SaturateOnIntegerOverflow=on
  Add2 : Sum  Inputs=++-  OutDataTypeStr=FOC_Fixed_Config.Types.Work  AccumDataTypeStr=FOC_Fixed_Config.Types.Work  RndMeth=Convergent  SaturateOnIntegerOverflow=on
  Constant : Constant  Value=FOC_Fixed_Config.Coefficients.psi.quantized  OutDataTypeStr=FOC_Fixed_Config.Types.Work
  Gain : Gain  Gain=FOC_Fixed_Config.Coefficients.Kaw_q.quantized  ParamDataTypeStr=FOC_Fixed_Config.Types.Coefficient  OutDataTypeStr=FOC_Fixed_Config.Types.Work  RndMeth=Convergent  SaturateOnIntegerOverflow=on
  Ld : Constant  Value=FOC_Fixed_Config.Coefficients.Ld.quantized  OutDataTypeStr=FOC_Fixed_Config.Types.Work
  Product : Product  OutDataTypeStr=FOC_Fixed_Config.Types.Work  RndMeth=Convergent  SaturateOnIntegerOverflow=on
  Product1 : Product  OutDataTypeStr=FOC_Fixed_Config.Types.Work  RndMeth=Convergent  SaturateOnIntegerOverflow=on
  Reset_Integral : Switch  Criteria=u2 > Threshold  Threshold=0.5  OutDataTypeStr=FOC_Fixed_Config.Types.Work  RndMeth=Convergent  InputSameDT=off
  Reset_Output : Switch  Criteria=u2 > Threshold  Threshold=0.5  OutDataTypeStr=FOC_Fixed_Config.Types.Work  RndMeth=Convergent  InputSameDT=off
  Reset_Zero : Constant  Value=0  OutDataTypeStr=FOC_Fixed_Config.Types.Work
  Sum : Sum  Inputs=|+-  OutDataTypeStr=FOC_Fixed_Config.Types.Work  AccumDataTypeStr=FOC_Fixed_Config.Types.Work  RndMeth=Convergent  SaturateOnIntegerOverflow=on
  Sum1 : Sum  Inputs=|++  OutDataTypeStr=FOC_Fixed_Config.Types.Work  AccumDataTypeStr=FOC_Fixed_Config.Types.Work  RndMeth=Convergent  SaturateOnIntegerOverflow=on
  x_q_z : UnitDelay  SampleTime=-1
  uq_raw : Outport
  wires:
  Iq_ref/1 -> Sum/1
  [x_q_next] -> x_q_z/1
  [du_q_z] -> Gain/1
  du_q_z/1 -> [du_q_z]
  "  "/1 -> Add1/1  "uq_p"
  Sum/1 -> " "/1, "  "/1  "e_q"
  Add/1 -> Product1/1
  Constant/1 -> Add/2
  Product/1 -> Add/1
  Ld/1 -> Product/2
  id/1 -> Product/1
  iq/1 -> Sum/2
  we/1 -> Product1/2
  Reset_Output/1 -> uq_raw/1
  Reset_Integral/1 -> [x_q_next]
  PI_Reset_EN/1 -> Reset_Output/2, Reset_Integral/2
  Reset_Zero/1 -> Reset_Output/1, Reset_Integral/1
  Add2/1 -> Reset_Integral/3  "x_q_next"
  Sum1/1 -> Reset_Output/3
  x_q_z/1 -> Add2/1, Add1/2
  " "/1 -> Add2/2  "KiTs_q * e_q"
  Gain/1 -> Add2/3  "u_q,aw"
  Add1/1 -> Sum1/1
  Product1/1 -> Sum1/2  "Ed"

== system gm_PMLSM_FOC_FixedPoint_vnl/FOC_DUT_vnl/SVPWMG ==
  Valpha : Inport
  Vbeta : Inport  Port=2
  Vdc_V : Inport  Port=3
  Duty Calculate : Subsystem  TreatAsAtomicUnit=on  RTWFcnName=Duty_Caculate_Fun
      settings: RTWFcnNameOpts=User specified
  Sector Caculate : Subsystem  TreatAsAtomicUnit=on  RTWFcnName=Sector_Caculate_Fun
      settings: RTWFcnNameOpts=User specified
  T1T2 Calculate : Subsystem  TreatAsAtomicUnit=on  RTWFcnName=T1T2Caculate_Fun
      settings: RTWFcnNameOpts=User specified
  XYZ Calculate : Subsystem  TreatAsAtomicUnit=on  RTWFcnName=XYZ_Caculate_Fun
      settings: RTWFcnNameOpts=User specified
  duty_u_cmd : Outport
  duty_v_cmd : Outport  Port=2
  duty_w_cmd : Outport  Port=3
  "N " : Outport  Port=4
  wires:
  Vdc_V/1 -> XYZ Calculate/3(Udc)
  Duty Calculate/3(Duty_W) -> duty_w_cmd/1
  Duty Calculate/2(Duty_V) -> duty_v_cmd/1
  Duty Calculate/1(Duty_U) -> duty_u_cmd/1
  XYZ Calculate/3(Z) -> T1T2 Calculate/4(Z)
  XYZ Calculate/2(Y) -> T1T2 Calculate/3(Y)
  XYZ Calculate/1(X) -> T1T2 Calculate/2(X)
  Sector Caculate/1("N ") -> T1T2 Calculate/1(N), Duty Calculate/1(N), "N "/1
  T1T2 Calculate/2(T2) -> Duty Calculate/3(T2)
  Valpha/1 -> XYZ Calculate/1(Ualpha), Sector Caculate/1(Ualpha)
  T1T2 Calculate/1(T1) -> Duty Calculate/2(T1)
  Vbeta/1 -> XYZ Calculate/2(Ubeta), Sector Caculate/2(Ubeta)

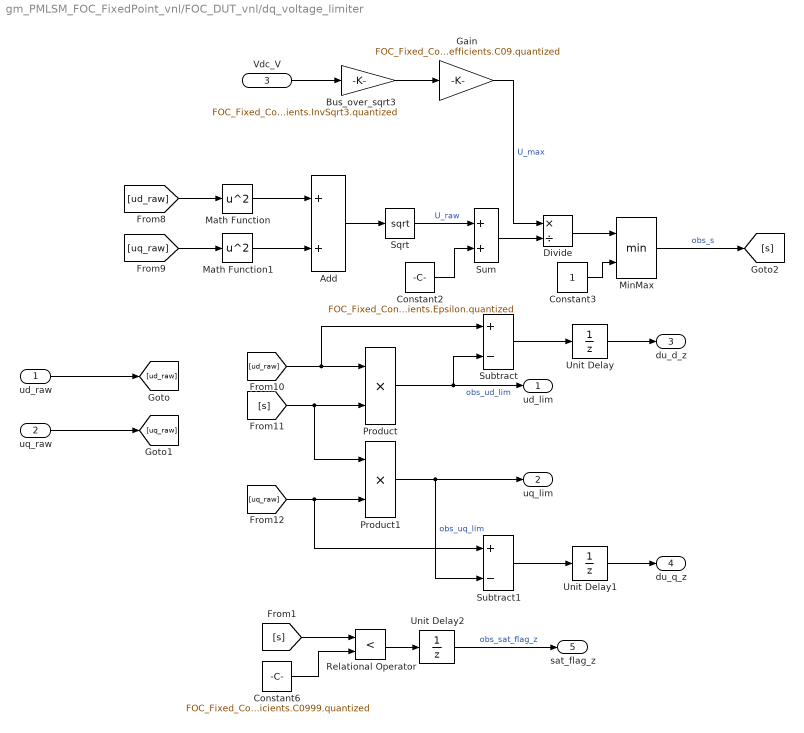
== system gm_PMLSM_FOC_FixedPoint_vnl/FOC_DUT_vnl/dq_voltage_limiter ==
  ud_raw : Inport
  uq_raw : Inport  Port=2
  Vdc_V : Inport  Port=3
  Add : Sum  OutDataTypeStr=FOC_Fixed_Config.Types.Square  AccumDataTypeStr=FOC_Fixed_Config.Types.Square  RndMeth=Convergent  SaturateOnIntegerOverflow=on
  Bus_over_sqrt3 : Gain  Gain=FOC_Fixed_Config.Coefficients.InvSqrt3.quantized  ParamDataTypeStr=FOC_Fixed_Config.Types.Coefficient  OutDataTypeStr=FOC_Fixed_Config.Types.Work  RndMeth=Convergent  SaturateOnIntegerOverflow=on
  Constant2 : Constant  Value=FOC_Fixed_Config.Coefficients.Epsilon.quantized  OutDataTypeStr=FOC_Fixed_Config.Types.Work
  Constant3 : Constant  OutDataTypeStr=FOC_Fixed_Config.Types.Work
  Constant6 : Constant  Value=FOC_Fixed_Config.Coefficients.C0999.quantized  OutDataTypeStr=FOC_Fixed_Config.Types.Work
  Divide : Product  Inputs=*/  OutDataTypeStr=FOC_Fixed_Config.Types.DivideWide  RndMeth=Convergent  SaturateOnIntegerOverflow=on
  Gain : Gain  Gain=FOC_Fixed_Config.Coefficients.C09.quantized  ParamDataTypeStr=FOC_Fixed_Config.Types.Coefficient  OutDataTypeStr=FOC_Fixed_Config.Types.Work  RndMeth=Convergent  SaturateOnIntegerOverflow=on
  Math Function : Math  Operator=square  OutDataTypeStr=FOC_Fixed_Config.Types.Square  RndMeth=Convergent
  Math Function1 : Math  Operator=square  OutDataTypeStr=FOC_Fixed_Config.Types.Square  RndMeth=Convergent
  MinMax : MinMax  Inputs=2  OutDataTypeStr=FOC_Fixed_Config.Types.Work  RndMeth=Convergent  SaturateOnIntegerOverflow=on
  Product : Product  OutDataTypeStr=FOC_Fixed_Config.Types.Work  RndMeth=Convergent  SaturateOnIntegerOverflow=on
  Product1 : Product  OutDataTypeStr=FOC_Fixed_Config.Types.Work  RndMeth=Convergent  SaturateOnIntegerOverflow=on
  Relational Operator : RelationalOperator  Operator=<  OutDataTypeStr=boolean  RndMeth=Convergent  InputSameDT=off
  Sqrt : Sqrt  OutDataTypeStr=FOC_Fixed_Config.Types.Work
  Subtract : Sum  Inputs=+-  OutDataTypeStr=FOC_Fixed_Config.Types.Work  AccumDataTypeStr=FOC_Fixed_Config.Types.Work  RndMeth=Convergent  SaturateOnIntegerOverflow=on
  Subtract1 : Sum  Inputs=+-  OutDataTypeStr=FOC_Fixed_Config.Types.Work  AccumDataTypeStr=FOC_Fixed_Config.Types.Work  RndMeth=Convergent  SaturateOnIntegerOverflow=on
  Sum : Sum  OutDataTypeStr=FOC_Fixed_Config.Types.Work  AccumDataTypeStr=FOC_Fixed_Config.Types.Work  RndMeth=Convergent  SaturateOnIntegerOverflow=on
  Unit Delay : UnitDelay  SampleTime=-1
  Unit Delay1 : UnitDelay  SampleTime=-1
  Unit Delay2 : UnitDelay  SampleTime=-1
  ud_lim : Outport
  uq_lim : Outport  Port=2
  du_d_z : Outport  Port=3
  du_q_z : Outport  Port=4
  sat_flag_z : Outport  Port=5
  wires:
  Gain/1 -> Divide/1  "U_max"
  Bus_over_sqrt3/1 -> Gain/1
  Vdc_V/1 -> Bus_over_sqrt3/1
  Unit Delay2/1 -> sat_flag_z/1  "obs_sat_flag_z"
  Relational Operator/1 -> Unit Delay2/1
  [s] -> Relational Operator/1
  Constant6/1 -> Relational Operator/2
  Unit Delay1/1 -> du_q_z/1
  Unit Delay/1 -> du_d_z/1
  uq_raw/1 -> [uq_raw]
  ud_raw/1 -> [ud_raw]
  Subtract1/1 -> Unit Delay1/1
  Subtract/1 -> Unit Delay/1
  [uq_raw] -> Product1/2, Subtract1/1
  Product/1 -> ud_lim/1, Subtract/2  "obs_ud_lim"
  [ud_raw] -> Product/1, Subtract/1
  [s] -> Product/2, Product1/1
  Product1/1 -> Subtract1/2, uq_lim/1  "obs_uq_lim"
  MinMax/1 -> [s]  "obs_s"
  [ud_raw] -> Math Function/1
  [uq_raw] -> Math Function1/1
  Math Function/1 -> Add/1
  Math Function1/1 -> Add/2
  Sqrt/1 -> Sum/1  "U_raw"
  Divide/1 -> MinMax/1
  Add/1 -> Sqrt/1
  Constant3/1 -> MinMax/2
  Constant2/1 -> Sum/2
  Sum/1 -> Divide/2

== system gm_PMLSM_FOC_FixedPoint_vnl/FOC_DUT/FOC_DUT/Clark ==
  ia : Inport  OutDataTypeStr=fixdt(1, 32, 24)  PortDimensions=1  SampleTime=2e-08
  ib : Inport  Port=2  OutDataTypeStr=fixdt(1, 32, 24)  PortDimensions=1  SampleTime=2e-08
  ic : Inport  Port=3  OutDataTypeStr=fixdt(1, 32, 24)  PortDimensions=1  SampleTime=2e-08
  Add1 : Sum  Inputs=+-  OutDataTypeStr=fixdt(1, 64, 40)  AccumDataTypeStr=fixdt(1, 64, 40)  RndMeth=Convergent  SaturateOnIntegerOverflow=on  SampleTime=2e-08
  Add_stage2 : Sum  Inputs=+-  OutDataTypeStr=fixdt(1, 64, 40)  AccumDataTypeStr=fixdt(1, 64, 40)  RndMeth=Convergent  SaturateOnIntegerOverflow=on  SampleTime=2e-08
  Add_stage3 : Sum  Inputs=+-  OutDataTypeStr=fixdt(1, 64, 40)  AccumDataTypeStr=fixdt(1, 64, 40)  RndMeth=Convergent  SaturateOnIntegerOverflow=on  SampleTime=2e-08
  Gain : Gain  Gain="fi(0,1,64,40,\"hex\",\"0000008000000000\")"  ParamDataTypeStr=fixdt(1, 64, 40)  OutDataTypeStr=fixdt(1, 64, 40)  RndMeth=Convergent  SaturateOnIntegerOverflow=on  SampleTime=2e-08
  Gain1 : Gain  Gain="fi(0,1,64,40,\"hex\",\"0000008000000000\")"  ParamDataTypeStr=fixdt(1, 64, 40)  OutDataTypeStr=fixdt(1, 64, 40)  RndMeth=Convergent  SaturateOnIntegerOverflow=on  SampleTime=2e-08
  Gain2 : Gain  Gain="fi(0,1,64,40,\"hex\",\"000000aaaaaaaaab\")"  ParamDataTypeStr=fixdt(1, 64, 40)  OutDataTypeStr=fixdt(1, 128, 80)  SampleTime=2e-08
  Gain2_out_dtc : DataTypeConversion  OutDataTypeStr=fixdt(1, 64, 40)  RndMeth=Convergent  SampleTime=2e-08
  Gain3 : Gain  Gain="fi(0,1,64,40,\"hex\",\"00000093cd3a2c82\")"  ParamDataTypeStr=fixdt(1, 64, 40)  OutDataTypeStr=fixdt(1, 128, 80)  SampleTime=2e-08
  Gain3_out_dtc : DataTypeConversion  OutDataTypeStr=fixdt(1, 64, 40)  RndMeth=Convergent  SampleTime=2e-08
  ialpha : Outport  OutDataTypeStr=fixdt(1, 64, 40)  PortDimensions=1  SampleTime=2e-08
  ibeta : Outport  Port=2  OutDataTypeStr=fixdt(1, 64, 40)  PortDimensions=1  SampleTime=2e-08
  wires:
  Gain2_out_dtc/1 -> ialpha/1
  Gain2/1 -> Gain2_out_dtc/1
  Gain3_out_dtc/1 -> ibeta/1
  Add_stage3/1 -> Gain2/1
  Gain3/1 -> Gain3_out_dtc/1
  Add_stage2/1 -> Add_stage3/1
  ia/1 -> Add_stage2/1
  Gain/1 -> Add_stage2/2
  ic/1 -> Add1/2, Gain1/1
  Add1/1 -> Gain3/1
  ib/1 -> Gain/1, Add1/1
  Gain1/1 -> Add_stage3/2

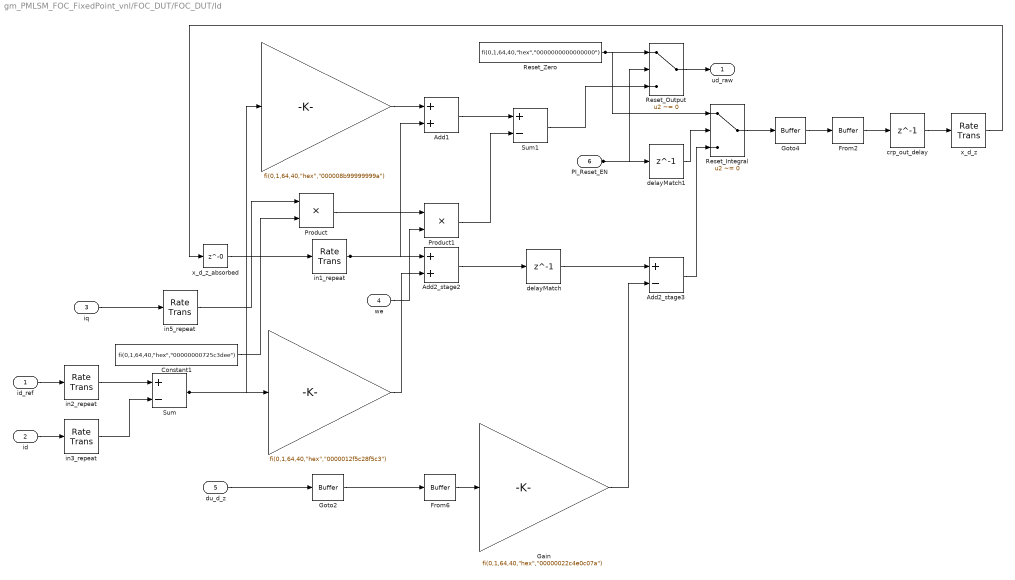
== system gm_PMLSM_FOC_FixedPoint_vnl/FOC_DUT/FOC_DUT/Id ==
  id_ref : Inport  OutDataTypeStr=fixdt(1, 32, 24)  PortDimensions=1  SampleTime=0.0001
  id : Inport  Port=2  OutDataTypeStr=fixdt(1, 64, 40)  PortDimensions=1  SampleTime=0.0001
  iq : Inport  Port=3  OutDataTypeStr=fixdt(1, 64, 40)  PortDimensions=1  SampleTime=0.0001
  we : Inport  Port=4  OutDataTypeStr=fixdt(1, 40, 24)  PortDimensions=1  SampleTime=2e-08
  du_d_z : Inport  Port=5  OutDataTypeStr=fixdt(1, 64, 40)  PortDimensions=1  SampleTime=2e-08
  PI_Reset_EN : Inport  Port=6  OutDataTypeStr=boolean  PortDimensions=1  SampleTime=2e-08
  " " : Gain  Gain="fi(0,1,64,40,\"hex\",\"0000012f5c28f5c3\")"  ParamDataTypeStr=fixdt(1, 64, 40)  OutDataTypeStr=fixdt(1, 64, 40)  RndMeth=Convergent  SaturateOnIntegerOverflow=on  SampleTime=2e-08
  "  " : Gain  Gain="fi(0,1,64,40,\"hex\",\"000008b99999999a\")"  ParamDataTypeStr=fixdt(1, 64, 40)  OutDataTypeStr=fixdt(1, 64, 40)  RndMeth=Convergent  SaturateOnIntegerOverflow=on  SampleTime=2e-08
  Add1 : Sum  OutDataTypeStr=fixdt(1, 64, 40)  AccumDataTypeStr=fixdt(1, 64, 40)  RndMeth=Convergent  SaturateOnIntegerOverflow=on  SampleTime=2e-08
  Add2_stage2 : Sum  OutDataTypeStr=fixdt(1, 64, 40)  AccumDataTypeStr=fixdt(1, 64, 40)  RndMeth=Convergent  SaturateOnIntegerOverflow=on  SampleTime=2e-08
  Add2_stage3 : Sum  Inputs=+-  OutDataTypeStr=fixdt(1, 64, 40)  AccumDataTypeStr=fixdt(1, 64, 40)  RndMeth=Convergent  SaturateOnIntegerOverflow=on  SampleTime=2e-08
  Constant1 : Constant  Value="fi(0,1,64,40,\"hex\",\"00000000725c3dee\")"  OutDataTypeStr=fixdt(1, 64, 40)  SampleTime=2e-08
  From2 : hdlmdlgenlib/Buffer
  From6 : hdlmdlgenlib/Buffer
  Gain : Gain  Gain="fi(0,1,64,40,\"hex\",\"00000022c4e0c07a\")"  ParamDataTypeStr=fixdt(1, 64, 40)  OutDataTypeStr=fixdt(1, 64, 40)  RndMeth=Convergent  SaturateOnIntegerOverflow=on  SampleTime=2e-08
  Goto2 : hdlmdlgenlib/Buffer
  Goto4 : hdlmdlgenlib/Buffer
  Product : Product  Inputs=**  OutDataTypeStr=fixdt(1, 64, 40)  RndMeth=Convergent  SaturateOnIntegerOverflow=on  SampleTime=2e-08
  Product1 : Product  Inputs=**  OutDataTypeStr=fixdt(1, 64, 40)  RndMeth=Convergent  SaturateOnIntegerOverflow=on  SampleTime=2e-08
  Reset_Integral : Switch  Criteria=u2 ~= 0  Threshold="fi(0,0,1,0,\"hex\",\"0\")"  OutDataTypeStr=fixdt(1, 64, 40)  RndMeth=Convergent  SampleTime=2e-08  InputSameDT=off
  Reset_Output : Switch  Criteria=u2 ~= 0  Threshold="fi(0,0,1,0,\"hex\",\"0\")"  OutDataTypeStr=fixdt(1, 64, 40)  RndMeth=Convergent  SampleTime=2e-08  InputSameDT=off
  Reset_Zero : Constant  Value="fi(0,1,64,40,\"hex\",\"0000000000000000\")"  OutDataTypeStr=fixdt(1, 64, 40)  SampleTime=2e-08
  Sum : Sum  Inputs=+-  OutDataTypeStr=fixdt(1, 64, 40)  AccumDataTypeStr=fixdt(1, 64, 40)  RndMeth=Convergent  SaturateOnIntegerOverflow=on  SampleTime=2e-08
  Sum1 : Sum  Inputs=+-  OutDataTypeStr=fixdt(1, 64, 40)  AccumDataTypeStr=fixdt(1, 64, 40)  RndMeth=Convergent  SaturateOnIntegerOverflow=on  SampleTime=2e-08
  crp_out_delay : Delay  DelayLength=1  InitialCondition=0  SampleTime=2e-08
  delayMatch : Delay  DelayLength=1  InitialCondition=0  SampleTime=2e-08
  delayMatch1 : Delay  DelayLength=1  InitialCondition=0  SampleTime=2e-08
  in1_repeat : RateTransition  Integrity=off  Deterministic=off  OutPortSampleTimeOpt=Multiple of input port sample time  OutPortSampleTimeMultiple=1/5000
  in2_repeat : RateTransition  Integrity=off  Deterministic=off  OutPortSampleTimeOpt=Multiple of input port sample time  OutPortSampleTimeMultiple=1/5000
  in3_repeat : RateTransition  Integrity=off  Deterministic=off  OutPortSampleTimeOpt=Multiple of input port sample time  OutPortSampleTimeMultiple=1/5000
  in5_repeat : RateTransition  Integrity=off  Deterministic=off  OutPortSampleTimeOpt=Multiple of input port sample time  OutPortSampleTimeMultiple=1/5000
  x_d_z : RateTransition  OutPortSampleTimeOpt=Multiple of input port sample time  OutPortSampleTimeMultiple=5000
  x_d_z_absorbed : Delay  DelayLength=0
  ud_raw : Outport  OutDataTypeStr=fixdt(1, 64, 40)  PortDimensions=1  SampleTime=2e-08
  wires:
  crp_out_delay/1 -> x_d_z/1
  From2/1 -> crp_out_delay/1
  Goto4/1 -> From2/1
  Reset_Integral/1 -> Goto4/1
  Add2_stage3/1 -> Reset_Integral/3
  delayMatch1/1 -> Reset_Integral/2
  Reset_Output/1 -> ud_raw/1
  Gain/1 -> Add2_stage3/2
  x_d_z/1 -> x_d_z_absorbed/1
  delayMatch/1 -> Add2_stage3/1
  Sum1/1 -> Reset_Output/3
  Reset_Zero/1 -> Reset_Output/1, Reset_Integral/1
  PI_Reset_EN/1 -> Reset_Output/2, delayMatch1/1
  Add2_stage2/1 -> delayMatch/1
  Add1/1 -> Sum1/1
  " "/1 -> Add2_stage2/2
  in1_repeat/1 -> Add2_stage2/1, Add1/2
  Product/1 -> Product1/1
  "  "/1 -> Add1/1
  du_d_z/1 -> Goto2/1
  Product1/1 -> Sum1/2
  Sum/1 -> " "/1, "  "/1
  we/1 -> Product1/2
  Constant1/1 -> Product/2
  in2_repeat/1 -> Sum/1
  iq/1 -> in5_repeat/1
  in3_repeat/1 -> Sum/2
  id/1 -> in3_repeat/1
  x_d_z_absorbed/1 -> in1_repeat/1
  id_ref/1 -> in2_repeat/1
  in5_repeat/1 -> Product/1
  Goto2/1 -> From6/1
  From6/1 -> Gain/1

== system gm_PMLSM_FOC_FixedPoint_vnl/FOC_DUT/FOC_DUT/InversePark ==
  A : Inport  OutDataTypeStr=fixdt(1,64,40,'DataTypeOverride', 'Off')  PortDimensions=1  SampleTime=2e-08
  B : Inport  Port=2  OutDataTypeStr=fixdt(1,64,40,'DataTypeOverride', 'Off')  PortDimensions=1  SampleTime=2e-08
  C : Inport  Port=3  OutDataTypeStr=fixdt(1,40,32,'DataTypeOverride', 'Off')  PortDimensions=1  SampleTime=0.0001
  Variant : Subsystem
  O1 : Outport  OutDataTypeStr=fixdt(1, 64, 40)  PortDimensions=1  SampleTime=2e-08
  O2 : Outport  Port=2  OutDataTypeStr=fixdt(1, 64, 40)  PortDimensions=1  SampleTime=2e-08
  wires:
  Variant/2(O2) -> O2/1
  Variant/1(O1) -> O1/1
  C/1 -> Variant/3(C)
  B/1 -> Variant/2(B)
  A/1 -> Variant/1(A)
